simulink model "dual_thyristor_bridge_rectifier"  (R2025b)
settings: Solver=ode1be  StartTime=0.0  StopTime=simlength  FixedStep=tc  MaxStep=tc
values from neighbouring files (symbols this model uses):
  n1 = 35    [voltage_spectrum_analysis.m]
  omega_grid_emulator_nom = w_grid    (= 314.159265359)    [grid_emulator.m]
  vn_eta_pu = 0    [grid_emulator.m]
  vn_xi_pu = 0    [grid_emulator.m]
  vp_xi_pu = 1    [grid_emulator.m]
  w_grid = f_grid*2*pi    (= 314.159265359)    [grid_emulator.m]
undefined symbols (not defined in the file or in its folder): CSF_11, CSF_13, CSF_5, CSF_7, delta_fht1, Idc_traction_normalization_factor, ki_u_ctrl, kp_u_ctrl, Ld_fht1, LFu_dc, LSF_11, LSF_13, LSF_5, LSF_7, magnitude, n10, omega_fht1, pll_i1, pll_p, RLFu_dc, tc, Tcontrol_rect, ts_ctrl_rect, ugrid_factor, Vdc_traction_normalization_factor, Vgrid_phase_normalization_factor
libraries: fl_lib x299, nesl_utility x67, ee_lib x24, single_phase_transformer_lib x3, cstblocks x3
(part 2 of 6)

== system dual_thyristor_bridge_rectifier/grid/grid_emulator ==
  3ph_Dyg : Subsystem
  Controlled Voltage Source : fl_lib/Electrical/Electrical Sources/Controlled Voltage Source
  Controlled Voltage Source1 : fl_lib/Electrical/Electrical Sources/Controlled Voltage Source
  Controlled Voltage Source2 : fl_lib/Electrical/Electrical Sources/Controlled Voltage Source
  Electrical Reference : fl_lib/Electrical/Electrical Elements/Electrical Reference
  Simulink-PS Converter : nesl_utility/Simulink-PS Converter  PhysicalDomain=network_engine_domain  SubClassName=ps_input  LeftPortType=input  RightPortType=output  PseudoPeriodic=off  Frequencies=[]  NoiseDistribution=none  NoiseParameters=[]  Unit=V  AffineConversion=on  FilteringAndDerivatives=provide  SimscapeFilterOrder=1  InputFilterTimeConstant=0.001  UdotUserProvided=0
  Simulink-PS Converter1 : nesl_utility/Simulink-PS Converter  PhysicalDomain=network_engine_domain  SubClassName=ps_input  LeftPortType=input  RightPortType=output  PseudoPeriodic=off  Frequencies=[]  NoiseDistribution=none  NoiseParameters=[]  Unit=V  AffineConversion=on  FilteringAndDerivatives=provide  SimscapeFilterOrder=1  InputFilterTimeConstant=0.001  UdotUserProvided=0
  Simulink-PS Converter2 : nesl_utility/Simulink-PS Converter  PhysicalDomain=network_engine_domain  SubClassName=ps_input  LeftPortType=input  RightPortType=output  PseudoPeriodic=off  Frequencies=[]  NoiseDistribution=none  NoiseParameters=[]  Unit=V  AffineConversion=on  FilteringAndDerivatives=provide  SimscapeFilterOrder=1  InputFilterTimeConstant=0.001  UdotUserProvided=0
  Solver Configuration : nesl_utility/Solver Configuration  PhysicalDomain=network_engine_domain  SubClassName=solver  LeftPortType=input  RightPortType=generic  Tones=[]  Harmonics=[]  SimulateNoise=off  Profile=off  UseLocalSampling=off  EnableSwitchedLinearOptims=on  FrequencyDomain=off  UseCCode=off  RelTol=0.001  AbsTol=0.001  MinStep=1e-09  ToWorkspace=off  RevertToSquareIcSolve=off  NumHomotopyIterations=100  PhasorMode=off  PhasorModeNumHarmonics=1  ConsistencySolver=NEWTON_FTOL  IndexReductionMethod=DerivativeReplacement  DoDC=off  ResidualTolerance=1e-09  ConsistencyTolSource=GLOBAL  ConsistencyAbsTol=0.001  ConsistencyRelTol=0.001  ConsistencyTolFactor=0.001  UseLocalSolver=on  LocalSolverChoice=NE_BACKWARD_EULER_ADVANCER  ResolveIndetEquations=on  FunctionEvalNumThread=1  LocalSolverSampleTime=tc  DoFixedCost=on  MaxNonlinIter=3  MaxModeIter=2  ComputeImpulses=off  ImpulseIterations=2  LinearAlgebra=auto  LinearAlgebraNumThread=0  EquationFormulation=NE_TIME_EF  DelaysMemoryBudget=1024  AutomaticFiltering=on  FilteringTimeConstant=0.001  PartitionStorageMethod=AS_NEEDED  PartitionMemoryBudget=1024  PartitionMethod=ROBUST  MultibodyUseLocalSolver=off  MultibodyLocalSolverChoice=ODE1  MultibodyLocalSolverSampleTime=0.001
  grid_emulator : Subsystem
  threephase_vi_measures : Subsystem
  u1 : PMIOPort  Side=Right
  u2 : PMIOPort  Port=2  Side=Right
  u3 : PMIOPort  Port=3  Side=Right
  wires:
  grid_emulator/2(Vmb) -> Simulink-PS Converter1/1
  grid_emulator/3(Vmc) -> Simulink-PS Converter2/1
  grid_emulator/1(Vma) -> Simulink-PS Converter/1
  connections:
  Simulink-PS Converter/RConn1 -- Controlled Voltage Source/RConn1
  Simulink-PS Converter1/RConn1 -- Controlled Voltage Source1/RConn1
  Simulink-PS Converter2/RConn1 -- Controlled Voltage Source2/RConn1
  Electrical Reference/LConn1 -- Solver Configuration/RConn1 -- Controlled Voltage Source/RConn2 -- Controlled Voltage Source1/RConn2 -- Controlled Voltage Source2/RConn2
  Controlled Voltage Source/LConn1 -- threephase_vi_measures/LConn1
  Controlled Voltage Source1/LConn1 -- threephase_vi_measures/LConn2
  Controlled Voltage Source2/LConn1 -- threephase_vi_measures/LConn3
  3ph_Dyg/LConn1 -- threephase_vi_measures/RConn1
  3ph_Dyg/LConn2 -- threephase_vi_measures/RConn2
  3ph_Dyg/LConn3 -- threephase_vi_measures/RConn3
  u2/RConn1 -- 3ph_Dyg/RConn2
  u1/RConn1 -- 3ph_Dyg/RConn1
  u3/RConn1 -- 3ph_Dyg/RConn3

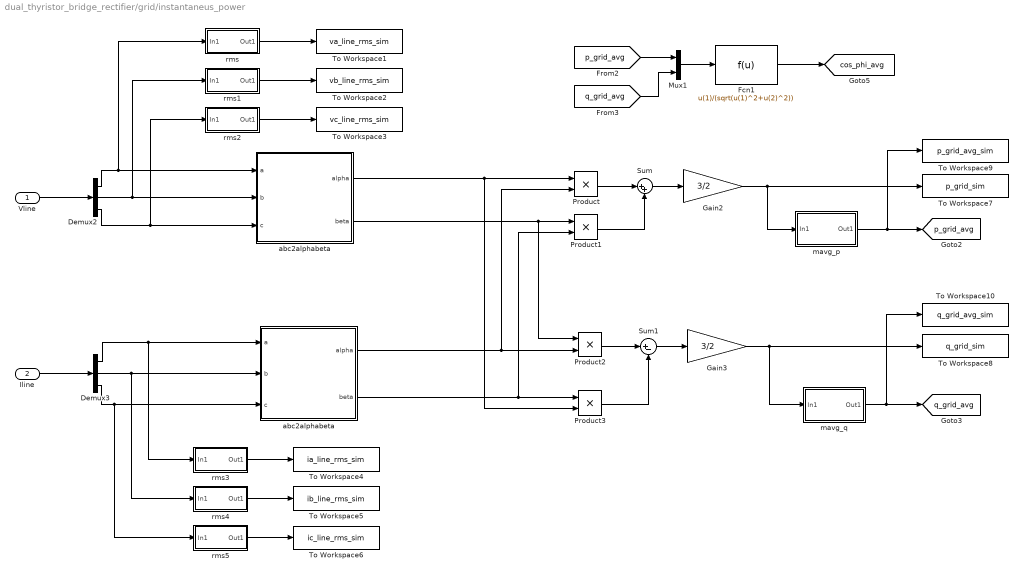
== system dual_thyristor_bridge_rectifier/grid/instantaneus_power ==
  Vline : Inport
  Iline : Inport  Port=2
  Demux2 : Demux  Outputs=3
  Demux3 : Demux  Outputs=3
  Fcn1 : Fcn  Expr=u(1)/(sqrt(u(1)^2+u(2)^2))
  Gain2 : Gain  Gain=3/2
  Gain3 : Gain  Gain=3/2
  Mux1 : Mux  Inputs=2
  Product{,1..3} (4 alike) : Product  RndMeth=Zero
  Sum : Sum  Inputs=|++
  Sum1 : Sum  Inputs=|+-
  To Workspace1 : ToWorkspace  VariableName=va_line_rms_sim  SampleTime=ts_ctrl_rect
      settings: MaxDataPoints=Ns_ctrl_rect
  To Workspace10 : ToWorkspace  VariableName=q_grid_avg_sim  SampleTime=ts_ctrl_rect
      settings: MaxDataPoints=Ns_ctrl_rect
  To Workspace2 : ToWorkspace  VariableName=vb_line_rms_sim  SampleTime=ts_ctrl_rect
      settings: MaxDataPoints=Ns_ctrl_rect
  To Workspace3 : ToWorkspace  VariableName=vc_line_rms_sim  SampleTime=ts_ctrl_rect
      settings: MaxDataPoints=Ns_ctrl_rect
  To Workspace4 : ToWorkspace  VariableName=ia_line_rms_sim  SampleTime=ts_ctrl_rect
      settings: MaxDataPoints=Ns_ctrl_rect
  To Workspace5 : ToWorkspace  VariableName=ib_line_rms_sim  SampleTime=ts_ctrl_rect
      settings: MaxDataPoints=Ns_ctrl_rect
  To Workspace6 : ToWorkspace  VariableName=ic_line_rms_sim  SampleTime=ts_ctrl_rect
      settings: MaxDataPoints=Ns_ctrl_rect
  To Workspace7 : ToWorkspace  VariableName=p_grid_sim  SampleTime=ts_ctrl_rect
      settings: MaxDataPoints=Ns_ctrl_rect
  To Workspace8 : ToWorkspace  VariableName=q_grid_sim  SampleTime=ts_ctrl_rect
      settings: MaxDataPoints=Ns_ctrl_rect
  To Workspace9 : ToWorkspace  VariableName=p_grid_avg_sim  SampleTime=ts_ctrl_rect
      settings: MaxDataPoints=Ns_ctrl_rect
  abc2alphabeta : Subsystem
  "abc2alphabeta " : Subsystem
  mavg_p : Subsystem
  mavg_q : Subsystem
  rms : Subsystem
  rms1 : Subsystem
  rms2 : Subsystem
  rms3 : Subsystem
  rms4 : Subsystem
  rms5 : Subsystem
  tag scope: cos_phi_avg=global, p_grid_avg=global, q_grid_avg=global
  wires:
  Gain3/1 -> mavg_q/1(In1), To Workspace8/1
  Demux2/1 -> abc2alphabeta/1(a), rms/1(In1)
  Vline/1 -> Demux2/1
  Iline/1 -> Demux3/1
  abc2alphabeta/2("beta ") -> Product1/1, Product2/1
  "abc2alphabeta "/2("beta ") -> Product3/1, Product1/2
  abc2alphabeta/1("alpha ") -> Product/1, Product3/2
  "abc2alphabeta "/1("alpha ") -> Product2/2, Product/2
  Product/1 -> Sum/1
  Product1/1 -> Sum/2
  Product2/1 -> Sum1/1
  Product3/1 -> Sum1/2
  Sum1/1 -> Gain3/1
  Sum/1 -> Gain2/1
  Demux2/2 -> abc2alphabeta/2(b), rms1/1(In1)
  Demux2/3 -> abc2alphabeta/3(c), rms2/1(In1)
  Demux3/1 -> rms3/1(In1), "abc2alphabeta "/1(a)
  Demux3/2 -> rms4/1(In1), "abc2alphabeta "/2(b)
  Demux3/3 -> rms5/1(In1), "abc2alphabeta "/3(c)
  Gain2/1 -> mavg_p/1(In1), To Workspace7/1
  mavg_q/1(Out1) -> To Workspace10/1, [q_grid_avg]
  [q_grid_avg] -> Mux1/2
  Mux1/1 -> Fcn1/1
  Fcn1/1 -> [cos_phi_avg]
  [p_grid_avg] -> Mux1/1
  rms/1(Out1) -> To Workspace1/1
  rms2/1(Out1) -> To Workspace3/1
  rms1/1(Out1) -> To Workspace2/1
  rms5/1(Out1) -> To Workspace6/1
  rms4/1(Out1) -> To Workspace5/1
  rms3/1(Out1) -> To Workspace4/1
  mavg_p/1(Out1) -> [p_grid_avg], To Workspace9/1

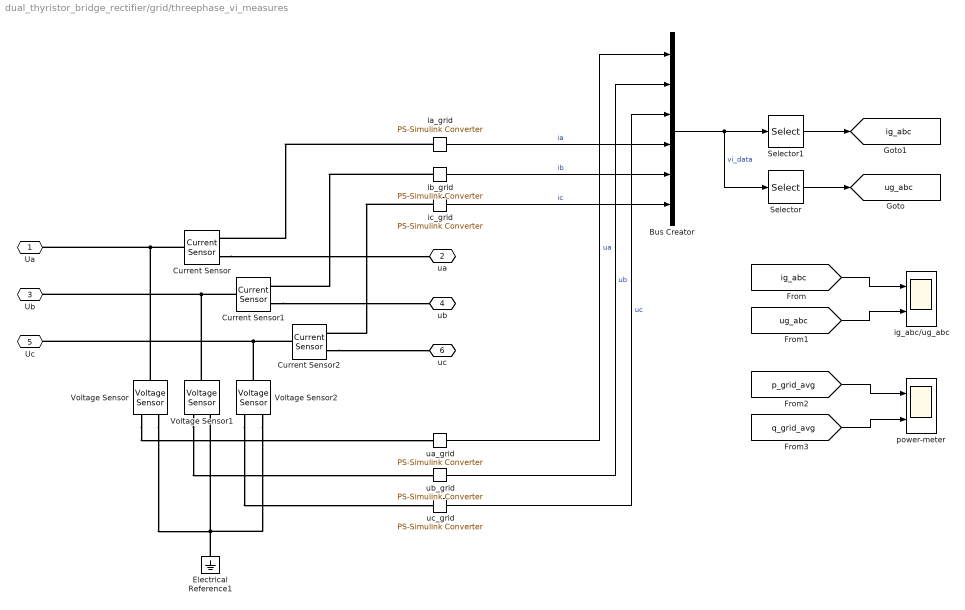
== system dual_thyristor_bridge_rectifier/grid/threephase_vi_measures ==
  Bus Creator : BusCreator  Inputs=6
  Current Sensor : fl_lib/Electrical/Electrical Sensors/Current Sensor
  Current Sensor1 : fl_lib/Electrical/Electrical Sensors/Current Sensor
  Current Sensor2 : fl_lib/Electrical/Electrical Sensors/Current Sensor
  Electrical Reference1 : fl_lib/Electrical/Electrical Elements/Electrical Reference
  Selector : Selector  InputPortWidth=6  IndexOptions=Index vector (dialog)  Indices=[1 2 3]  OutputSizes=1
  Selector1 : Selector  InputPortWidth=6  IndexOptions=Index vector (dialog)  Indices=[4 5 6]  OutputSizes=1
  Voltage Sensor : fl_lib/Electrical/Electrical Sensors/Voltage Sensor
  Voltage Sensor1 : fl_lib/Electrical/Electrical Sensors/Voltage Sensor
  Voltage Sensor2 : fl_lib/Electrical/Electrical Sensors/Voltage Sensor
  ia_grid : nesl_utility/PS-Simulink Converter  PhysicalDomain=network_engine_domain  SubClassName=ps_output  LeftPortType=input  RightPortType=output  PseudoPeriodic=off  Frequencies=[]  VectorFormat=1-D array  Unit=A  AffineConversion=off
  ib_grid : nesl_utility/PS-Simulink Converter  PhysicalDomain=network_engine_domain  SubClassName=ps_output  LeftPortType=input  RightPortType=output  PseudoPeriodic=off  Frequencies=[]  VectorFormat=1-D array  Unit=A  AffineConversion=off
  ic_grid : nesl_utility/PS-Simulink Converter  PhysicalDomain=network_engine_domain  SubClassName=ps_output  LeftPortType=input  RightPortType=output  PseudoPeriodic=off  Frequencies=[]  VectorFormat=1-D array  Unit=A  AffineConversion=off
  ig_abc/ug_abc : Scope  NumInputPorts=2
      settings: SampleTime=tc  ActiveDisplayYMinimum=-3558.44602  ActiveDisplayYMaximum=3125.9197  DataLoggingVariableName=ScopeData2
  power-meter : Scope  NumInputPorts=2
      settings: SampleTime=tc  ActiveDisplayYMinimum=-110289.50474  ActiveDisplayYMaximum=992605.54264  DataLoggingVariableName=ScopeData3
  ua_grid : nesl_utility/PS-Simulink Converter  PhysicalDomain=network_engine_domain  SubClassName=ps_output  LeftPortType=input  RightPortType=output  PseudoPeriodic=off  Frequencies=[]  VectorFormat=1-D array  Unit=V  AffineConversion=off
  ub_grid : nesl_utility/PS-Simulink Converter  PhysicalDomain=network_engine_domain  SubClassName=ps_output  LeftPortType=input  RightPortType=output  PseudoPeriodic=off  Frequencies=[]  VectorFormat=1-D array  Unit=V  AffineConversion=off
  uc_grid : nesl_utility/PS-Simulink Converter  PhysicalDomain=network_engine_domain  SubClassName=ps_output  LeftPortType=input  RightPortType=output  PseudoPeriodic=off  Frequencies=[]  VectorFormat=1-D array  Unit=V  AffineConversion=off
  Ua : PMIOPort  Side=Left
  ua : PMIOPort  Port=2  Side=Right
  Ub : PMIOPort  Port=3  Side=Left
  ub : PMIOPort  Port=4  Side=Right
  Uc : PMIOPort  Port=5  Side=Left
  uc : PMIOPort  Port=6  Side=Right
  tag scope: ig_abc=global, ug_abc=global
  wires:
  Bus Creator/1 -> Selector1/1, Selector/1  "vi_data"
  Selector/1 -> [ug_abc]
  ib_grid/1 -> Bus Creator/5  "ib"
  ia_grid/1 -> Bus Creator/4  "ia"
  ic_grid/1 -> Bus Creator/6  "ic"
  ua_grid/1 -> Bus Creator/1  "ua"
  ub_grid/1 -> Bus Creator/2  "ub"
  uc_grid/1 -> Bus Creator/3  "uc"
  Selector1/1 -> [ig_abc]
  [ug_abc] -> ig_abc/ug_abc/2
  [ig_abc] -> ig_abc/ug_abc/1
  [p_grid_avg] -> power-meter/1
  [q_grid_avg] -> power-meter/2
  connections:
  Current Sensor1/LConn1 -- Ub/RConn1 -- Voltage Sensor1/LConn1
  Electrical Reference1/LConn1 -- Voltage Sensor/RConn2 -- Voltage Sensor2/RConn2 -- Voltage Sensor1/RConn2
  Voltage Sensor/RConn1 -- ua_grid/LConn1
  Current Sensor/RConn2 -- ua/RConn1
  Voltage Sensor1/RConn1 -- ub_grid/LConn1
  Voltage Sensor2/LConn1 -- Current Sensor2/LConn1 -- Uc/RConn1
  Current Sensor/LConn1 -- Ua/RConn1 -- Voltage Sensor/LConn1
  Current Sensor1/RConn2 -- ub/RConn1
  Voltage Sensor2/RConn1 -- uc_grid/LConn1
  ib_grid/LConn1 -- Current Sensor1/RConn1
  ia_grid/LConn1 -- Current Sensor/RConn1
  ic_grid/LConn1 -- Current Sensor2/RConn1
  Current Sensor2/RConn2 -- uc/RConn1

== system dual_thyristor_bridge_rectifier/load_and_control/controller ==
  Constant1 : Constant  Value=5
  Constant2 : Constant
  Constant3 : Constant  Value=1000
  Constant4 : Constant  Value=25
  MATLAB Function1 : MATLAB Function  TreatAsAtomicUnit=on  SystemSampleTime=ts_ctrl_rect
  Unit Delay1 : UnitDelay  SampleTime=ts_ctrl_rect  HasFrameUpgradeWarning=on
  Unit Delay2 : UnitDelay  SampleTime=ts_ctrl_rect  HasFrameUpgradeWarning=on
  Zero-Order Hold : ZeroOrderHold  SampleTime=ts_ctrl_rect
  Zero-Order Hold1 : ZeroOrderHold  SampleTime=ts_ctrl_rect
  firing_angle & switches : Scope  NumInputPorts=4
      settings: SampleTime=ts  ActiveDisplayYMinimum=-0.5  ActiveDisplayYMaximum=4.5  DataLoggingVariableName=ScopeData2
  firing_angles : Scope  NumInputPorts=3
      settings: SampleTime=ts  ActiveDisplayYMinimum=-0.3802  ActiveDisplayYMaximum=3.42179
  pi_voltage_ctrl : Subsystem
  tag scope: enable_neg_bridge=global, enable_pos_bridge=global, firing_angle=global, pi_voltage_ctrl_output=global, reg_fsm_state=global
  wires:
  [u_out] -> pi_voltage_ctrl/2(vout)
  Constant2/1 -> pi_voltage_ctrl/1(vout_ref)
  [i_out] -> Zero-Order Hold/1
  Constant1/1 -> MATLAB Function1/4(i_th1)
  MATLAB Function1/1(pos) -> firing_angle & switches/2, [enable_pos_bridge]  "enable_pos_bridge"
  Unit Delay2/1 -> MATLAB Function1/3(i)
  Zero-Order Hold/1 -> Unit Delay2/1
  [u_out] -> Zero-Order Hold1/1
  Zero-Order Hold1/1 -> Unit Delay1/1
  Unit Delay1/1 -> MATLAB Function1/1(u)
  Constant3/1 -> MATLAB Function1/2(u_th)
  MATLAB Function1/3(alpha_out) -> firing_angle & switches/1, firing_angles/1, [firing_angle]  "firing_angle"
  pi_voltage_ctrl/1(w) -> MATLAB Function1/6(alpha_in), firing_angles/3, [pi_voltage_ctrl_output]  "pi_voltage_ctrl_output"
  MATLAB Function1/2(neg) -> firing_angles/2, firing_angle & switches/3, [enable_neg_bridge]  "enable_neg_bridge"
  Constant4/1 -> MATLAB Function1/5(i_th2)
  MATLAB Function1/4(state_out) -> firing_angle & switches/4, [reg_fsm_state]  "state"

== system dual_thyristor_bridge_rectifier/dual_rectifier_bridge/C-caller ctrl/Subsystem2 ==
  "PD " : Inport
  Bus Selector : BusSelector  OutputSignals=pd_1,pd_2,pd_3,pd_4,pd_5,pd_6
  Data Type Conversion{1..6} (6 alike) : DataTypeConversion  OutDataTypeStr=double  SaturateOnIntegerOverflow=off  RndMeth=Floor
  Gain{,1..5} (6 alike) : Gain  Gain=12
  Mux : Mux  Inputs=6
  Rate Transition{,1..5} (6 alike) : RateTransition  OutPortSampleTime=ts
  PD : Outport
  wires:
  Bus Selector/3 -> Data Type Conversion2/1  "<pd_3>"
  Mux/1 -> PD/1
  Bus Selector/6 -> Data Type Conversion6/1  "<pd_6>"
  Bus Selector/1 -> Data Type Conversion5/1  "<pd_1>"
  Bus Selector/4 -> Data Type Conversion3/1  "<pd_4>"
  "PD "/1 -> Bus Selector/1
  Bus Selector/2 -> Data Type Conversion1/1  "<pd_2>"
  Bus Selector/5 -> Data Type Conversion4/1  "<pd_5>"
  Data Type Conversion5/1 -> Rate Transition/1
  Data Type Conversion1/1 -> Rate Transition1/1
  Data Type Conversion2/1 -> Rate Transition2/1
  Data Type Conversion3/1 -> Rate Transition3/1
  Data Type Conversion4/1 -> Rate Transition4/1
  Data Type Conversion6/1 -> Rate Transition5/1
  Gain/1 -> Mux/1
  Gain1/1 -> Mux/2
  Gain2/1 -> Mux/3
  Gain3/1 -> Mux/4
  Gain4/1 -> Mux/5
  Gain5/1 -> Mux/6
  Rate Transition/1 -> Gain/1
  Rate Transition1/1 -> Gain1/1
  Rate Transition2/1 -> Gain2/1
  Rate Transition3/1 -> Gain3/1
  Rate Transition4/1 -> Gain4/1
  Rate Transition5/1 -> Gain5/1

== system dual_thyristor_bridge_rectifier/dual_rectifier_bridge/C-caller ctrl/Subsystem3 ==
  "PY " : Inport
  Bus Selector : BusSelector  OutputSignals=py_1,py_2,py_3,py_4,py_5,py_6
  Data Type Conversion{,1..5} (6 alike) : DataTypeConversion  OutDataTypeStr=double  SaturateOnIntegerOverflow=off  RndMeth=Floor
  Gain{,1..5} (6 alike) : Gain  Gain=12
  Mux : Mux  Inputs=6
  Rate Transition{,1..5} (6 alike) : RateTransition  OutPortSampleTime=ts
  PY : Outport
  wires:
  Bus Selector/5 -> Data Type Conversion4/1  "<py_5>"
  Bus Selector/2 -> Data Type Conversion1/1  "<py_2>"
  "PY "/1 -> Bus Selector/1
  Bus Selector/4 -> Data Type Conversion3/1  "<py_4>"
  Bus Selector/1 -> Data Type Conversion/1  "<py_1>"
  Bus Selector/6 -> Data Type Conversion5/1  "<py_6>"
  Mux/1 -> PY/1
  Bus Selector/3 -> Data Type Conversion2/1  "<py_3>"
  Data Type Conversion/1 -> Rate Transition/1
  Data Type Conversion1/1 -> Rate Transition1/1
  Data Type Conversion2/1 -> Rate Transition2/1
  Data Type Conversion3/1 -> Rate Transition3/1
  Data Type Conversion4/1 -> Rate Transition4/1
  Data Type Conversion5/1 -> Rate Transition5/1
  Gain/1 -> Mux/1
  Gain1/1 -> Mux/2
  Gain2/1 -> Mux/3
  Gain3/1 -> Mux/4
  Gain4/1 -> Mux/5
  Gain5/1 -> Mux/6
  Rate Transition/1 -> Gain/1
  Rate Transition1/1 -> Gain1/1
  Rate Transition2/1 -> Gain2/1
  Rate Transition3/1 -> Gain3/1
  Rate Transition4/1 -> Gain4/1
  Rate Transition5/1 -> Gain5/1

== system dual_thyristor_bridge_rectifier/dual_rectifier_bridge/L_filter/shunt_passive_filter_11 ==
  Capacitor : fl_lib/Electrical/Electrical Elements/Capacitor  c=CSF F  r=RCSF Ohm  g=0 1/Ohm  i_specify=off  i_priority=None  i=0 A  i_nominal_specify=off  i_nominal_value=1  i_nominal_unit=A  v_specify=off  v_priority=None  v=0 V  v_nominal_specify=off  v_nominal_value=1  v_nominal_unit=V  vc_specify=off  vc_priority=High  vc=0 V  vc_nominal_specify=off  vc_nominal_value=1  vc_nominal_unit=V
  Capacitor1 : fl_lib/Electrical/Electrical Elements/Capacitor  c=CSF F  r=RCSF Ohm  g=0 1/Ohm  i_specify=off  i_priority=None  i=0 A  i_nominal_specify=off  i_nominal_value=1  i_nominal_unit=A  v_specify=off  v_priority=None  v=0 V  v_nominal_specify=off  v_nominal_value=1  v_nominal_unit=V  vc_specify=off  vc_priority=High  vc=0 V  vc_nominal_specify=off  vc_nominal_value=1  vc_nominal_unit=V
  Capacitor2 : fl_lib/Electrical/Electrical Elements/Capacitor  c=CSF F  r=RCSF Ohm  g=0 1/Ohm  i_specify=off  i_priority=None  i=0 A  i_nominal_specify=off  i_nominal_value=1  i_nominal_unit=A  v_specify=off  v_priority=None  v=0 V  v_nominal_specify=off  v_nominal_value=1  v_nominal_unit=V  vc_specify=off  vc_priority=High  vc=0 V  vc_nominal_specify=off  vc_nominal_value=1  vc_nominal_unit=V
  Current Sensor1 : fl_lib/Electrical/Electrical Sensors/Current Sensor
  Inductor1 : fl_lib/Electrical/Electrical Elements/Inductor  l=LSF H  r=0 Ohm  g=1e-9 1/Ohm  i_specify=on  i_priority=High  i=0 A  i_nominal_specify=off  i_nominal_value=1  i_nominal_unit=A  v_specify=off  v_priority=None  v=0 V  v_nominal_specify=off  v_nominal_value=1  v_nominal_unit=V  i_L_specify=off  i_L_priority=High  i_L=0 A  i_L_nominal_specify=off  i_L_nominal_value=1  i_L_nominal_unit=A
  Inductor2 : fl_lib/Electrical/Electrical Elements/Inductor  l=LSF H  r=0 Ohm  g=1e-9 1/Ohm  i_specify=on  i_priority=High  i=0 A  i_nominal_specify=off  i_nominal_value=1  i_nominal_unit=A  v_specify=off  v_priority=None  v=0 V  v_nominal_specify=off  v_nominal_value=1  v_nominal_unit=V  i_L_specify=off  i_L_priority=High  i_L=0 A  i_L_nominal_specify=off  i_L_nominal_value=1  i_L_nominal_unit=A
  Inductor3 : fl_lib/Electrical/Electrical Elements/Inductor  l=LSF H  r=0 Ohm  g=1e-9 1/Ohm  i_specify=on  i_priority=High  i=0 A  i_nominal_specify=off  i_nominal_value=1  i_nominal_unit=A  v_specify=off  v_priority=None  v=0 V  v_nominal_specify=off  v_nominal_value=1  v_nominal_unit=V  i_L_specify=off  i_L_priority=High  i_L=0 A  i_L_nominal_specify=off  i_L_nominal_value=1  i_L_nominal_unit=A
  PS-Simulink Converter2 : nesl_utility/PS-Simulink Converter  PhysicalDomain=network_engine_domain  SubClassName=ps_output  LeftPortType=input  RightPortType=output  PseudoPeriodic=off  Frequencies=[]  VectorFormat=1-D array  Unit=A  AffineConversion=off
  a : PMIOPort  Side=Right
  b : PMIOPort  Port=2  Side=Right
  c : PMIOPort  Port=3  Side=Right
  tag scope: ic_SF11=global
  wires:
  PS-Simulink Converter2/1 -> [ic_SF11]
  connections:
  Capacitor/LConn1 -- Inductor3/LConn1
  Capacitor1/LConn1 -- Inductor1/LConn1
  Inductor2/LConn1 -- Capacitor2/LConn1
  a/RConn1 -- Inductor3/RConn1 -- Inductor2/RConn1
  Inductor1/RConn1 -- Capacitor/RConn1 -- b/RConn1
  Capacitor1/RConn1 -- Current Sensor1/RConn2 -- c/RConn1
  Capacitor2/RConn1 -- Current Sensor1/LConn1
  PS-Simulink Converter2/LConn1 -- Current Sensor1/RConn1

== system dual_thyristor_bridge_rectifier/dual_rectifier_bridge/L_filter/shunt_passive_filter_13 ==
  Capacitor : fl_lib/Electrical/Electrical Elements/Capacitor  c=CSF F  r=RCSF Ohm  g=0 1/Ohm  i_specify=off  i_priority=None  i=0 A  i_nominal_specify=off  i_nominal_value=1  i_nominal_unit=A  v_specify=off  v_priority=None  v=0 V  v_nominal_specify=off  v_nominal_value=1  v_nominal_unit=V  vc_specify=off  vc_priority=High  vc=0 V  vc_nominal_specify=off  vc_nominal_value=1  vc_nominal_unit=V
  Capacitor1 : fl_lib/Electrical/Electrical Elements/Capacitor  c=CSF F  r=RCSF Ohm  g=0 1/Ohm  i_specify=off  i_priority=None  i=0 A  i_nominal_specify=off  i_nominal_value=1  i_nominal_unit=A  v_specify=off  v_priority=None  v=0 V  v_nominal_specify=off  v_nominal_value=1  v_nominal_unit=V  vc_specify=off  vc_priority=High  vc=0 V  vc_nominal_specify=off  vc_nominal_value=1  vc_nominal_unit=V
  Capacitor2 : fl_lib/Electrical/Electrical Elements/Capacitor  c=CSF F  r=RCSF Ohm  g=0 1/Ohm  i_specify=off  i_priority=None  i=0 A  i_nominal_specify=off  i_nominal_value=1  i_nominal_unit=A  v_specify=off  v_priority=None  v=0 V  v_nominal_specify=off  v_nominal_value=1  v_nominal_unit=V  vc_specify=off  vc_priority=High  vc=0 V  vc_nominal_specify=off  vc_nominal_value=1  vc_nominal_unit=V
  Current Sensor1 : fl_lib/Electrical/Electrical Sensors/Current Sensor
  Inductor1 : fl_lib/Electrical/Electrical Elements/Inductor  l=LSF H  r=0 Ohm  g=1e-9 1/Ohm  i_specify=on  i_priority=High  i=0 A  i_nominal_specify=off  i_nominal_value=1  i_nominal_unit=A  v_specify=off  v_priority=None  v=0 V  v_nominal_specify=off  v_nominal_value=1  v_nominal_unit=V  i_L_specify=off  i_L_priority=High  i_L=0 A  i_L_nominal_specify=off  i_L_nominal_value=1  i_L_nominal_unit=A
  Inductor2 : fl_lib/Electrical/Electrical Elements/Inductor  l=LSF H  r=0 Ohm  g=1e-9 1/Ohm  i_specify=on  i_priority=High  i=0 A  i_nominal_specify=off  i_nominal_value=1  i_nominal_unit=A  v_specify=off  v_priority=None  v=0 V  v_nominal_specify=off  v_nominal_value=1  v_nominal_unit=V  i_L_specify=off  i_L_priority=High  i_L=0 A  i_L_nominal_specify=off  i_L_nominal_value=1  i_L_nominal_unit=A
  Inductor3 : fl_lib/Electrical/Electrical Elements/Inductor  l=LSF H  r=0 Ohm  g=1e-9 1/Ohm  i_specify=on  i_priority=High  i=0 A  i_nominal_specify=off  i_nominal_value=1  i_nominal_unit=A  v_specify=off  v_priority=None  v=0 V  v_nominal_specify=off  v_nominal_value=1  v_nominal_unit=V  i_L_specify=off  i_L_priority=High  i_L=0 A  i_L_nominal_specify=off  i_L_nominal_value=1  i_L_nominal_unit=A
  PS-Simulink Converter2 : nesl_utility/PS-Simulink Converter  PhysicalDomain=network_engine_domain  SubClassName=ps_output  LeftPortType=input  RightPortType=output  PseudoPeriodic=off  Frequencies=[]  VectorFormat=1-D array  Unit=A  AffineConversion=off
  a : PMIOPort  Side=Right
  b : PMIOPort  Port=2  Side=Right
  c : PMIOPort  Port=3  Side=Right
  tag scope: ic_SF13=global
  wires:
  PS-Simulink Converter2/1 -> [ic_SF13]
  connections:
  Capacitor1/RConn1 -- c/RConn1 -- Current Sensor1/RConn2
  b/RConn1 -- Capacitor/RConn1 -- Inductor1/RConn1
  Inductor2/RConn1 -- Inductor3/RConn1 -- a/RConn1
  Inductor2/LConn1 -- Capacitor2/LConn1
  Capacitor1/LConn1 -- Inductor1/LConn1
  Capacitor/LConn1 -- Inductor3/LConn1
  Capacitor2/RConn1 -- Current Sensor1/LConn1
  PS-Simulink Converter2/LConn1 -- Current Sensor1/RConn1

== system dual_thyristor_bridge_rectifier/dual_rectifier_bridge/L_filter/shunt_passive_filter_5 ==
  Capacitor : fl_lib/Electrical/Electrical Elements/Capacitor  c=CSF F  r=RCSF Ohm  g=0 1/Ohm  i_specify=off  i_priority=None  i=0 A  i_nominal_specify=off  i_nominal_value=1  i_nominal_unit=A  v_specify=off  v_priority=None  v=0 V  v_nominal_specify=off  v_nominal_value=1  v_nominal_unit=V  vc_specify=off  vc_priority=High  vc=0 V  vc_nominal_specify=off  vc_nominal_value=1  vc_nominal_unit=V
  Capacitor1 : fl_lib/Electrical/Electrical Elements/Capacitor  c=CSF F  r=RCSF Ohm  g=0 1/Ohm  i_specify=off  i_priority=None  i=0 A  i_nominal_specify=off  i_nominal_value=1  i_nominal_unit=A  v_specify=off  v_priority=None  v=0 V  v_nominal_specify=off  v_nominal_value=1  v_nominal_unit=V  vc_specify=off  vc_priority=High  vc=0 V  vc_nominal_specify=off  vc_nominal_value=1  vc_nominal_unit=V
  Capacitor2 : fl_lib/Electrical/Electrical Elements/Capacitor  c=CSF F  r=RCSF Ohm  g=0 1/Ohm  i_specify=off  i_priority=None  i=0 A  i_nominal_specify=off  i_nominal_value=1  i_nominal_unit=A  v_specify=off  v_priority=None  v=0 V  v_nominal_specify=off  v_nominal_value=1  v_nominal_unit=V  vc_specify=off  vc_priority=High  vc=0 V  vc_nominal_specify=off  vc_nominal_value=1  vc_nominal_unit=V
  Current Sensor1 : fl_lib/Electrical/Electrical Sensors/Current Sensor
  Inductor1 : fl_lib/Electrical/Electrical Elements/Inductor  l=LSF H  r=0 Ohm  g=1e-9 1/Ohm  i_specify=on  i_priority=High  i=0 A  i_nominal_specify=off  i_nominal_value=1  i_nominal_unit=A  v_specify=off  v_priority=None  v=0 V  v_nominal_specify=off  v_nominal_value=1  v_nominal_unit=V  i_L_specify=off  i_L_priority=High  i_L=0 A  i_L_nominal_specify=off  i_L_nominal_value=1  i_L_nominal_unit=A
  Inductor2 : fl_lib/Electrical/Electrical Elements/Inductor  l=LSF H  r=0 Ohm  g=1e-9 1/Ohm  i_specify=on  i_priority=High  i=0 A  i_nominal_specify=off  i_nominal_value=1  i_nominal_unit=A  v_specify=off  v_priority=None  v=0 V  v_nominal_specify=off  v_nominal_value=1  v_nominal_unit=V  i_L_specify=off  i_L_priority=High  i_L=0 A  i_L_nominal_specify=off  i_L_nominal_value=1  i_L_nominal_unit=A
  Inductor3 : fl_lib/Electrical/Electrical Elements/Inductor  l=LSF H  r=0 Ohm  g=1e-9 1/Ohm  i_specify=on  i_priority=High  i=0 A  i_nominal_specify=off  i_nominal_value=1  i_nominal_unit=A  v_specify=off  v_priority=None  v=0 V  v_nominal_specify=off  v_nominal_value=1  v_nominal_unit=V  i_L_specify=off  i_L_priority=High  i_L=0 A  i_L_nominal_specify=off  i_L_nominal_value=1  i_L_nominal_unit=A
  PS-Simulink Converter2 : nesl_utility/PS-Simulink Converter  PhysicalDomain=network_engine_domain  SubClassName=ps_output  LeftPortType=input  RightPortType=output  PseudoPeriodic=off  Frequencies=[]  VectorFormat=1-D array  Unit=A  AffineConversion=off
  a : PMIOPort  Side=Right
  b : PMIOPort  Port=2  Side=Right
  c : PMIOPort  Port=3  Side=Right
  tag scope: ic_SF5=global
  wires:
  PS-Simulink Converter2/1 -> [ic_SF5]
  connections:
  Capacitor/LConn1 -- Inductor3/LConn1
  Capacitor1/LConn1 -- Inductor1/LConn1
  Inductor2/LConn1 -- Capacitor2/LConn1
  a/RConn1 -- Inductor2/RConn1 -- Inductor3/RConn1
  Capacitor/RConn1 -- b/RConn1 -- Inductor1/RConn1
  Capacitor1/RConn1 -- Current Sensor1/RConn2 -- c/RConn1
  Current Sensor1/LConn1 -- Capacitor2/RConn1
  PS-Simulink Converter2/LConn1 -- Current Sensor1/RConn1

== system dual_thyristor_bridge_rectifier/dual_rectifier_bridge/L_filter/shunt_passive_filter_7 ==
  Capacitor : fl_lib/Electrical/Electrical Elements/Capacitor  c=CSF F  r=RCSF Ohm  g=0 1/Ohm  i_specify=off  i_priority=None  i=0 A  i_nominal_specify=off  i_nominal_value=1  i_nominal_unit=A  v_specify=off  v_priority=None  v=0 V  v_nominal_specify=off  v_nominal_value=1  v_nominal_unit=V  vc_specify=off  vc_priority=High  vc=0 V  vc_nominal_specify=off  vc_nominal_value=1  vc_nominal_unit=V
  Capacitor1 : fl_lib/Electrical/Electrical Elements/Capacitor  c=CSF F  r=RCSF Ohm  g=0 1/Ohm  i_specify=off  i_priority=None  i=0 A  i_nominal_specify=off  i_nominal_value=1  i_nominal_unit=A  v_specify=off  v_priority=None  v=0 V  v_nominal_specify=off  v_nominal_value=1  v_nominal_unit=V  vc_specify=off  vc_priority=High  vc=0 V  vc_nominal_specify=off  vc_nominal_value=1  vc_nominal_unit=V
  Capacitor2 : fl_lib/Electrical/Electrical Elements/Capacitor  c=CSF F  r=RCSF Ohm  g=0 1/Ohm  i_specify=off  i_priority=None  i=0 A  i_nominal_specify=off  i_nominal_value=1  i_nominal_unit=A  v_specify=off  v_priority=None  v=0 V  v_nominal_specify=off  v_nominal_value=1  v_nominal_unit=V  vc_specify=off  vc_priority=High  vc=0 V  vc_nominal_specify=off  vc_nominal_value=1  vc_nominal_unit=V
  Current Sensor1 : fl_lib/Electrical/Electrical Sensors/Current Sensor
  Inductor1 : fl_lib/Electrical/Electrical Elements/Inductor  l=LSF H  r=0 Ohm  g=1e-9 1/Ohm  i_specify=on  i_priority=High  i=0 A  i_nominal_specify=off  i_nominal_value=1  i_nominal_unit=A  v_specify=off  v_priority=None  v=0 V  v_nominal_specify=off  v_nominal_value=1  v_nominal_unit=V  i_L_specify=off  i_L_priority=High  i_L=0 A  i_L_nominal_specify=off  i_L_nominal_value=1  i_L_nominal_unit=A
  Inductor2 : fl_lib/Electrical/Electrical Elements/Inductor  l=LSF H  r=0 Ohm  g=1e-9 1/Ohm  i_specify=on  i_priority=High  i=0 A  i_nominal_specify=off  i_nominal_value=1  i_nominal_unit=A  v_specify=off  v_priority=None  v=0 V  v_nominal_specify=off  v_nominal_value=1  v_nominal_unit=V  i_L_specify=off  i_L_priority=High  i_L=0 A  i_L_nominal_specify=off  i_L_nominal_value=1  i_L_nominal_unit=A
  Inductor3 : fl_lib/Electrical/Electrical Elements/Inductor  l=LSF H  r=0 Ohm  g=1e-9 1/Ohm  i_specify=on  i_priority=High  i=0 A  i_nominal_specify=off  i_nominal_value=1  i_nominal_unit=A  v_specify=off  v_priority=None  v=0 V  v_nominal_specify=off  v_nominal_value=1  v_nominal_unit=V  i_L_specify=off  i_L_priority=High  i_L=0 A  i_L_nominal_specify=off  i_L_nominal_value=1  i_L_nominal_unit=A
  PS-Simulink Converter2 : nesl_utility/PS-Simulink Converter  PhysicalDomain=network_engine_domain  SubClassName=ps_output  LeftPortType=input  RightPortType=output  PseudoPeriodic=off  Frequencies=[]  VectorFormat=1-D array  Unit=A  AffineConversion=off
  a : PMIOPort  Side=Right
  b : PMIOPort  Port=2  Side=Right
  c : PMIOPort  Port=3  Side=Right
  tag scope: ic_SF7=global
  wires:
  PS-Simulink Converter2/1 -> [ic_SF7]
  connections:
  Capacitor1/RConn1 -- Current Sensor1/RConn2 -- c/RConn1
  b/RConn1 -- Capacitor/RConn1 -- Inductor1/RConn1
  Inductor2/RConn1 -- Inductor3/RConn1 -- a/RConn1
  Inductor2/LConn1 -- Capacitor2/LConn1
  Capacitor1/LConn1 -- Inductor1/LConn1
  Capacitor/LConn1 -- Inductor3/LConn1
  Capacitor2/RConn1 -- Current Sensor1/LConn1
  PS-Simulink Converter2/LConn1 -- Current Sensor1/RConn1

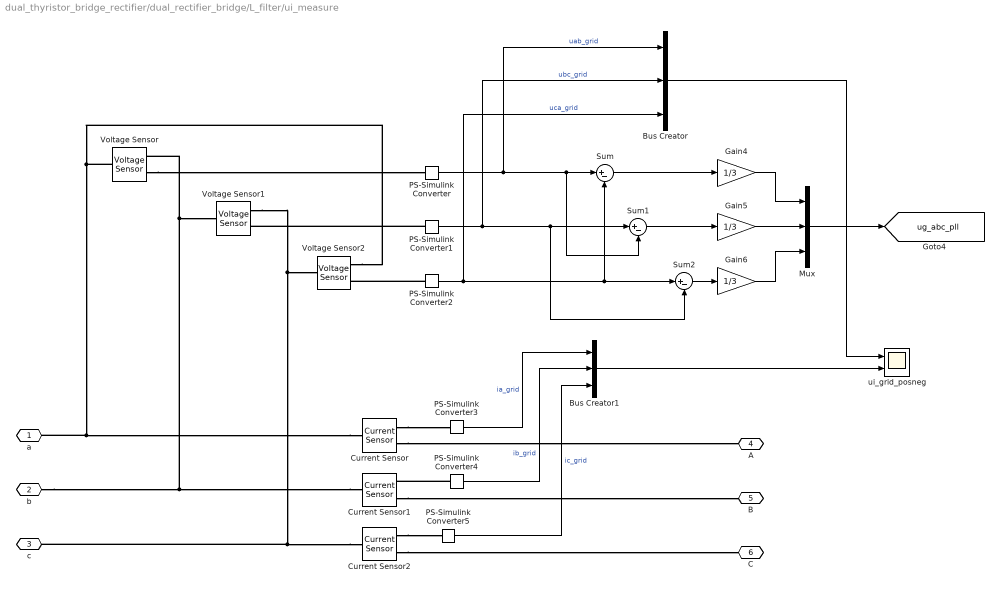
== system dual_thyristor_bridge_rectifier/dual_rectifier_bridge/L_filter/ui_measure ==
  Bus Creator : BusCreator  Inputs=3
  Bus Creator1 : BusCreator  Inputs=3
  Current Sensor : fl_lib/Electrical/Electrical Sensors/Current Sensor
  Current Sensor1 : fl_lib/Electrical/Electrical Sensors/Current Sensor
  Current Sensor2 : fl_lib/Electrical/Electrical Sensors/Current Sensor
  Gain4 : Gain  Gain=1/3
  Gain5 : Gain  Gain=1/3
  Gain6 : Gain  Gain=1/3
  Mux : Mux  Inputs=3
  PS-Simulink Converter : nesl_utility/PS-Simulink Converter  PhysicalDomain=network_engine_domain  SubClassName=ps_output  LeftPortType=input  RightPortType=output  PseudoPeriodic=off  Frequencies=[]  VectorFormat=1-D array  Unit=V  AffineConversion=off
  PS-Simulink Converter1 : nesl_utility/PS-Simulink Converter  PhysicalDomain=network_engine_domain  SubClassName=ps_output  LeftPortType=input  RightPortType=output  PseudoPeriodic=off  Frequencies=[]  VectorFormat=1-D array  Unit=V  AffineConversion=off
  PS-Simulink Converter2 : nesl_utility/PS-Simulink Converter  PhysicalDomain=network_engine_domain  SubClassName=ps_output  LeftPortType=input  RightPortType=output  PseudoPeriodic=off  Frequencies=[]  VectorFormat=1-D array  Unit=V  AffineConversion=off
  PS-Simulink Converter3 : nesl_utility/PS-Simulink Converter  PhysicalDomain=network_engine_domain  SubClassName=ps_output  LeftPortType=input  RightPortType=output  PseudoPeriodic=off  Frequencies=[]  VectorFormat=1-D array  Unit=A  AffineConversion=off
  PS-Simulink Converter4 : nesl_utility/PS-Simulink Converter  PhysicalDomain=network_engine_domain  SubClassName=ps_output  LeftPortType=input  RightPortType=output  PseudoPeriodic=off  Frequencies=[]  VectorFormat=1-D array  Unit=A  AffineConversion=off
  PS-Simulink Converter5 : nesl_utility/PS-Simulink Converter  PhysicalDomain=network_engine_domain  SubClassName=ps_output  LeftPortType=input  RightPortType=output  PseudoPeriodic=off  Frequencies=[]  VectorFormat=1-D array  Unit=A  AffineConversion=off
  Sum : Sum  Inputs=|+-
  Sum1 : Sum  Inputs=|+-
  Sum2 : Sum  Inputs=|+-
  Voltage Sensor : fl_lib/Electrical/Electrical Sensors/Voltage Sensor
  Voltage Sensor1 : fl_lib/Electrical/Electrical Sensors/Voltage Sensor
  Voltage Sensor2 : fl_lib/Electrical/Electrical Sensors/Voltage Sensor
  ui_grid_posneg : Scope  NumInputPorts=2
      settings: SampleTime=ts  ActiveDisplayYMinimum=-1547.89942  ActiveDisplayYMaximum=1487.26806
  a : PMIOPort  Side=Left
  b : PMIOPort  Port=2  Side=Left
  c : PMIOPort  Port=3  Side=Left
  A : PMIOPort  Port=4  Side=Right
  B : PMIOPort  Port=5  Side=Right
  C : PMIOPort  Port=6  Side=Right
  tag scope: ug_abc_pll=global
  wires:
  Bus Creator/1 -> ui_grid_posneg/1
  Bus Creator1/1 -> ui_grid_posneg/2
  PS-Simulink Converter5/1 -> Bus Creator1/3  "ic_grid"
  PS-Simulink Converter4/1 -> Bus Creator1/2  "ib_grid"
  PS-Simulink Converter3/1 -> Bus Creator1/1  "ia_grid"
  Sum2/1 -> Gain6/1
  Sum1/1 -> Gain5/1
  Sum/1 -> Gain4/1
  Gain5/1 -> Mux/2
  Gain4/1 -> Mux/1
  Gain6/1 -> Mux/3
  PS-Simulink Converter1/1 -> Sum1/1, Sum2/2, Bus Creator/2  "ubc_grid"
  PS-Simulink Converter2/1 -> Sum/2, Sum2/1, Bus Creator/3  "uca_grid"
  PS-Simulink Converter/1 -> Sum1/2, Sum/1, Bus Creator/1  "uab_grid"
  Mux/1 -> [ug_abc_pll]
  connections:
  Current Sensor/RConn2 -- A/RConn1
  Current Sensor1/RConn2 -- B/RConn1
  Current Sensor2/RConn2 -- C/RConn1
  Current Sensor2/RConn1 -- PS-Simulink Converter5/LConn1
  PS-Simulink Converter4/LConn1 -- Current Sensor1/RConn1
  Current Sensor/RConn1 -- PS-Simulink Converter3/LConn1
  PS-Simulink Converter2/LConn1 -- Voltage Sensor2/RConn1
  Current Sensor2/LConn1 -- Voltage Sensor2/LConn1 -- Voltage Sensor1/RConn2 -- c/RConn1
  PS-Simulink Converter1/LConn1 -- Voltage Sensor1/RConn1
  Voltage Sensor/RConn1 -- PS-Simulink Converter/LConn1
  Current Sensor1/LConn1 -- Voltage Sensor1/LConn1 -- Voltage Sensor/RConn2 -- b/RConn1
  Current Sensor/LConn1 -- Voltage Sensor/LConn1 -- Voltage Sensor2/RConn2 -- a/RConn1

== system dual_thyristor_bridge_rectifier/dual_rectifier_bridge/neg_bridge/firing1 ==
  Capacitor1 : fl_lib/Electrical/Electrical Elements/Capacitor  Commented=on  c=100e-6 F  r=1e-6 Ohm  g=0 1/Ohm  i_specify=off  i_priority=None  i=0 A  i_nominal_specify=off  i_nominal_value=1  i_nominal_unit=A  v_specify=off  v_priority=None  v=0 V  v_nominal_specify=off  v_nominal_value=1  v_nominal_unit=V  vc_specify=off  vc_priority=High  vc=0 V  vc_nominal_specify=off  vc_nominal_value=1  vc_nominal_unit=V
  Capacitor2 : fl_lib/Electrical/Electrical Elements/Capacitor  Commented=on  c=100e-12 F  r=1e-6 Ohm  g=0 1/Ohm  i_specify=off  i_priority=None  i=0 A  i_nominal_specify=off  i_nominal_value=1  i_nominal_unit=A  v_specify=off  v_priority=None  v=0 V  v_nominal_specify=off  v_nominal_value=1  v_nominal_unit=V  vc_specify=off  vc_priority=High  vc=0 V  vc_nominal_specify=off  vc_nominal_value=1  vc_nominal_unit=V
  Controlled Voltage Source1 : fl_lib/Electrical/Electrical Sources/Controlled Voltage Source  Commented=on
  Controlled Voltage Source2 : fl_lib/Electrical/Electrical Sources/Controlled Voltage Source  Commented=on
  Diode : fl_lib/Electrical/Electrical Elements/Diode  Commented=on  Vf=0.6 V  Ron=0.3 Ohm  Goff=1e-8 1/Ohm  i_specify=off  i_priority=None  i=0 A  i_nominal_specify=off  i_nominal_value=1  i_nominal_unit=A  v_specify=off  v_priority=None  v=0 V  v_nominal_specify=off  v_nominal_value=1  v_nominal_unit=V
  Diode2 : fl_lib/Electrical/Electrical Elements/Diode  Commented=on  Vf=0.6 V  Ron=0.3 Ohm  Goff=1e-8 1/Ohm  i_specify=off  i_priority=None  i=0 A  i_nominal_specify=off  i_nominal_value=1  i_nominal_unit=A  v_specify=off  v_priority=None  v=0 V  v_nominal_specify=off  v_nominal_value=1  v_nominal_unit=V
  Diode3 : fl_lib/Electrical/Electrical Elements/Diode  Commented=on  Vf=0.6 V  Ron=0.3 Ohm  Goff=1e-8 1/Ohm  i_specify=off  i_priority=None  i=0 A  i_nominal_specify=off  i_nominal_value=1  i_nominal_unit=A  v_specify=off  v_priority=None  v=0 V  v_nominal_specify=off  v_nominal_value=1  v_nominal_unit=V
  Electrical Reference3 : fl_lib/Electrical/Electrical Elements/Electrical Reference  Commented=on
  Electrical Reference4 : fl_lib/Electrical/Electrical Elements/Electrical Reference  Commented=on
  Electrical Reference5 : fl_lib/Electrical/Electrical Elements/Electrical Reference  Commented=on
  "IGBT (Ideal, Switching)" : ee_lib/Semiconductors & Converters/IGBT (Ideal, Switching)  Commented=on  port_option=ee.enum.controlport.elec  Vf=0.8 V  Ron=0.001 Ohm  Goff=1e-5 1/Ohm  Vth=2 V  diode_param=1  diode_Vf=0.8 V  diode_Ron=0.001 Ohm  diode_Goff=1e-5 1/Ohm  diode_C=50e-9 F  diode_iRM=-235 A  diode_iF=300 A  diode_idot=-50 A/us  diode_trr_param=1  diode_trr_factor=3  diode_trr=15 us  diode_Qrr=1500 s*uA  ice_specify=off  ice_priority=None  ice=0 A  ice_nominal_specify=off  ice_nominal_value=1  ice_nominal_unit=A  vce_specify=off  vce_priority=None  vce=0 V  vce_nominal_specify=off  vce_nominal_value=1  vce_nominal_unit=V  vge_specify=off  vge_priority=None  vge=0 V  vge_nominal_specify=off  vge_nominal_value=1  vge_nominal_unit=V  thermal_loss_option=2  Von_data=[0, 1.1, 1.3, 1.45, 1.75, 2.25, 2.7; 0, 1, 1.15, 1.35, 1.7, 2.35, 3] V  Tj=[298.15, 398.15] K  Iout_data=[0, 10, 50, 100, 200, 400, 600] A  Eon_data=[0, .29, 1.43, 2.86, 5.71, 13.14, 22.86; 0, .57, 2.63, 5.14, 10.29, 20.57, 30.29] * 1e-3 J  Eoff_data=[0, .21, 1.07, 2.14, 4.29, 9.86, 17.14; 0, .43, 1.97, 3.86, 7.71, 15.43, 22.71] * 1e-3 J  Eon_data_3D=[zeros(2, 9, 3)] J  Eoff_data_3D=[zeros(2, 9, 3)] J  Tj_loss=[298.15, 398.15] K  Iout_data_loss=[0, .1, 1, 5, 10, 20, 40, 70, 100] A  tabulateWithVce=false  Vce_loss=[0, 150, 300] V  Eon_scalar=22.86e-3 J  Eoff_scalar=17.14e-3 J  Voff=300 V  Iout_scalar=600 A  useCurrentFromPreviousCycle=false  useVoltageFromPreviousCycle=false  diodeModelType=ee.enum.converters.diodeModelType.pwl  diodeTableType=ee.enum.diode.tableType.IfMat  diode_ReverseIVType=ee.enum.diode.diodeReverseIV.constant  diode_IfMat=[.07, .12, .19, 1.75, 4.24, 7.32, 11.2; .16, .3, .72, 2.14, 4.02, 6.35, 9.12] A  diode_VfMat=[.9, 1.15, 1.25, 1.5, 1.75, 2.17, 2.6, 2.85; .58, .68, .75, 1.1, 1.38, 1.77, 2.27, 2.7] V  diode_TjVec=[25, 125] degC  diode_VfVec=[.5, .7, .9, 1.3, 1.7, 2.1, 2.5] V  diode_IfVec=[.1, .2, .5, 1, 2, 4, 7, 10] A  diode_IrMat=[1e-06, 2e-06, 5e-06, 1e-05, 2.5e-05, 5e-05, .0001; 2e-06, 5e-06, 1e-05, 4e-05, 8e-05, .0002, .0005] A  diode_VrMat=[10, 100, 200, 250, 300, 325, 350; 10, 70, 160, 220, 270, 300, 320] V  diode_VrVec=[10, 20, 40, 50, 70, 80, 100] V  diode_IrVec=[1e-06, 2e-06, 5e-06, 1e-05, 2e-05, 5e-05, .0001] A  diode_Vr=-600 V  diode_Ls=150 nH  diode_Erec=0.03 J  diode_rec_loss_model=ee.enum.diode.reverseRecoveryModel.fixed  diode_ErecVal=0 J  diode_scaleWithIandV=true  diode_ErecMat=zeros(2, 3) J  diode_TjrecVec=[298.15, 398.15] K  diode_IfrecVec=[.1, 1, 10] A  diode_IrecVal=10 A  diode_VrecVal=10 V  diode_tFilter=1 / 1000 / 100 s  separateThermalPortForDiode=false  thermal_network_parameterization=ee.enum.thermalNetworkTopology.external  Rth=[.08, .5] K/W  Rth_Cauer=[.08, .1, .5] K/W  Rth_Foster=[.08, .14, .22, .16] K/W  thermal_mass_parameterization=ee.enum.thermalNetwork.timeconstant  thermal_mass=[.01, .5] J/K  thermal_mass_Cauer=[.01, .1, .5] J/K  thermal_mass_Foster=[.001, .005, .05, .5] J/K  thermal_time_constant=[.001, .2] s  thermal_time_constant_Cauer=[.001, .1, .2] s  thermal_time_constant_Foster=[7e-05, .0007, .01, .08] s  thermal_mass_initial_temperatures=[25, 25] degC  thermal_mass_initial_temperatures_Cauer=[25, 25, 25] degC  junction_thermal_mass=0.01 J/K  Tvec_initial_Foster=[25, 25, 25, 25] degC  RthDiode=[.03, .2] K/W  RthCauerDiode=[.03, .1, .2] K/W  RthFosterDiode=[.03, .2] K/W  thermalMassDiode=[3, 25] J/K  thermalMassCauerDiode=[3, 10, 25] J/K  thermalMassFosterDiode=[33, 50] J/K  thermalTauDiode=[.1, 5] s  thermalTauCauerDiode=[.1, 1, 5] s  thermalTauFosterDiode=[1, 10] s  thermalMassInitTempDiode=[25, 25] degC  thermalMassInitTempCauerDiode=[25, 25, 25] degC  junctionthermalMassDiode=0.1 J/K  TVecInitialFosterDiode=[25, 25, 25, 25] degC  no_thermal_network=0  IGBT_junction_temperature_specify=off  IGBT_junction_temperature_priority=None  IGBT_junction_temperature=25 degC  IGBT_junction_temperature_nominal_specify=off  IGBT_junction_temperature_nominal_value=1  IGBT_junction_temperature_nominal_unit=degC  diode_junction_temperature_specify=off  diode_junction_temperature_priority=None  diode_junction_temperature=25 degC  diode_junction_temperature_nominal_specify=off  diode_junction_temperature_nominal_value=1  diode_junction_temperature_nominal_unit=degC  Qj_specify=off  Qj_priority=None  Qj=0 W  Qj_nominal_specify=off  Qj_nominal_value=1  Qj_nominal_unit=W  accumulatedSwitchingLosses_specify=off  accumulatedSwitchingLosses_priority=None  accumulatedSwitchingLosses=0 J
      settings: InternalSimscapePortConfiguration="{\"Bottom\":[],\"Left\":[{\"id\":\"G_elec\",\"label\":\"\",\"type\":\"foundation.electrical.electrical\"}],\"Right\":[{\"id\":\"C\",\"label\":\"\",\"type\":\"foundation.electrical.electrical\"},{\"id\":\"E\",\"label\":\"\",\"type\":\"foundation.electrical.electrical\"}],\"Top\":[]}"
  Ideal Transformer : fl_lib/Electrical/Electrical Elements/Ideal Transformer  Commented=on  n=2  i1_specify=off  i1_priority=None  i1=0 A  i1_nominal_specify=off  i1_nominal_value=1  i1_nominal_unit=A  v1_specify=off  v1_priority=None  v1=0 V  v1_nominal_specify=off  v1_nominal_value=1  v1_nominal_unit=V  i2_specify=off  i2_priority=None  i2=0 A  i2_nominal_specify=off  i2_nominal_value=1  i2_nominal_unit=A  v2_specify=off  v2_priority=None  v2=0 V  v2_nominal_specify=off  v2_nominal_value=1  v2_nominal_unit=V
  PS Constant : fl_lib/Physical Signals/Sources/PS Constant  Commented=on  constant=48 V
  Resistor1 : fl_lib/Electrical/Electrical Elements/Resistor  Commented=on  R=470 Ohm  i_specify=off  i_priority=None  i=0 A  i_nominal_specify=off  i_nominal_value=1  i_nominal_unit=A  v_specify=off  v_priority=None  v=0 V  v_nominal_specify=off  v_nominal_value=1  v_nominal_unit=V
  Resistor3 : fl_lib/Electrical/Electrical Elements/Resistor  Commented=on  R=470 Ohm  i_specify=off  i_priority=None  i=0 A  i_nominal_specify=off  i_nominal_value=1  i_nominal_unit=A  v_specify=off  v_priority=None  v=0 V  v_nominal_specify=off  v_nominal_value=1  v_nominal_unit=V
  Resistor5 : fl_lib/Electrical/Electrical Elements/Resistor  Commented=on  R=100 Ohm  i_specify=off  i_priority=None  i=0 A  i_nominal_specify=off  i_nominal_value=1  i_nominal_unit=A  v_specify=off  v_priority=None  v=0 V  v_nominal_specify=off  v_nominal_value=1  v_nominal_unit=V
  Resistor6 : fl_lib/Electrical/Electrical Elements/Resistor  Commented=on  R=1e9 Ohm  i_specify=off  i_priority=None  i=0 A  i_nominal_specify=off  i_nominal_value=1  i_nominal_unit=A  v_specify=off  v_priority=None  v=0 V  v_nominal_specify=off  v_nominal_value=1  v_nominal_unit=V
  Voltage Sensor : fl_lib/Electrical/Electrical Sensors/Voltage Sensor  Commented=on
  oscillator : Subsystem  Commented=on
  gin : PMIOPort  Side=Left
  g+ : PMIOPort  Port=2  Side=Right
  connections:
  Resistor3/LConn1 -- Controlled Voltage Source1/LConn1
  Electrical Reference5/LConn1 -- Capacitor1/RConn1
  Capacitor1/LConn1 -- Resistor3/RConn1 -- Diode3/LConn1
  "IGBT (Ideal, Switching)"/RConn1 -- Diode3/RConn1
  Resistor6/RConn1 -- Electrical Reference3/LConn1
  PS Constant/RConn1 -- Controlled Voltage Source1/RConn1
  Capacitor2/LConn1 -- Voltage Sensor/LConn1 -- Resistor5/LConn1 -- Diode2/RConn1
  Resistor5/RConn1 -- Resistor6/LConn1 -- Ideal Transformer/RConn2 -- Voltage Sensor/RConn2 -- Capacitor2/RConn1
  Ideal Transformer/RConn1 -- Diode2/LConn1
  Diode/RConn1 -- Ideal Transformer/LConn1 -- "IGBT (Ideal, Switching)"/RConn2 -- Controlled Voltage Source1/RConn2 -- Controlled Voltage Source2/RConn2
  Controlled Voltage Source2/LConn1 -- Resistor1/LConn1
  Ideal Transformer/LConn2 -- Diode/LConn1 -- Electrical Reference4/LConn1
  "IGBT (Ideal, Switching)"/LConn1 -- Resistor1/RConn1
  gin/RConn1 -- g+/RConn1
